simulink model "timedSpikingTestOpt2"  (R2026b)
settings: Solver=FixedStepAuto  StopTime=15  FixedStep=0.001
libraries: simulink x1, dspsigops x1
settings Model: Creator=40129232  LastModifiedBy=Eoin
settings DataIOCC: ReturnWorkspaceOutputs=off
settings OptimizationCC: LifeSpan=inf
settings DebuggingCC: ArithmeticOperatorsInVariantConditions=warning  SFExecutionAtInitializationDiag=none
settings SFSimCC: CustomCodeUndefinedFunction=UseInterfaceOnly  SimUseLocalCustomCode=off
settings RTWCC: DLArmComputeVersion=19.05  RTWUseLocalCustomCode=off
settings CodeAppCC: StateflowObjectComments=on

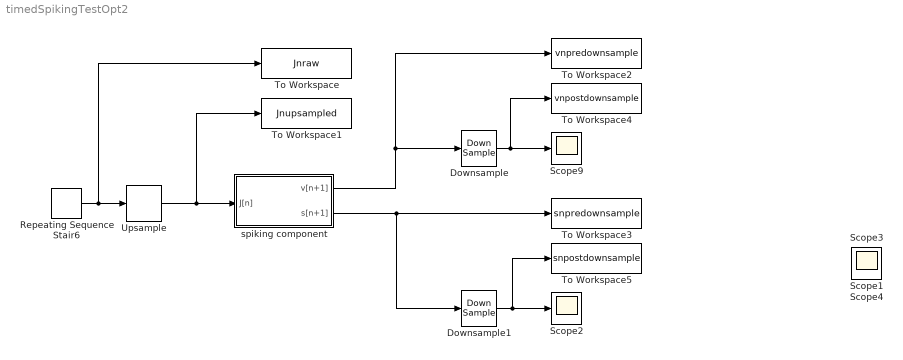
== system timedSpikingTestOpt2 ==
  Downsample : DownSample  DownsamplingFactor=15
  Downsample1 : DownSample  DownsamplingFactor=15
  Repeating Sequence Stair6 : simulink/Sources/Repeating Sequence Stair  OutValues=[40.37, 52.35, 62.17, 70.19, 76.75].'  tsamp=0.015  OutMin=[]  OutMax=[]  OutDataTypeStr=double  OutputDataTypeScalingMode=double  OutDataType=fixdt(0,8)  ConRadixGroup=Best Precision: Vector-wise  OutScaling=2^-12
  Scope{1..4,9} (5 alike) : Scope
      Scope2 settings: ActiveDisplayYMinimum=-0.36753410515202733  ActiveDisplayYMaximum=1.2278178479729731
      Scope9 settings: ActiveDisplayYMinimum=-91.1513790892599  ActiveDisplayYMaximum=42.518602095331268  DataLoggingVariableName=ScopeData5
      Scope1 settings: ActiveDisplayYMinimum=-0.24987  ActiveDisplayYMaximum=2.24887
      Scope3 settings: ActiveDisplayYMinimum=-103.72127  ActiveDisplayYMaximum=38.33358  DataLoggingVariableName=ScopeData3
      Scope4 settings: ActiveDisplayYMinimum=-20.75486  ActiveDisplayYMaximum=56.79378  DataLoggingVariableName=ScopeData4
  To Workspace : ToWorkspace  VariableName=Jnraw  SaveFormat=Timeseries  SampleTime=-1
  To Workspace1 : ToWorkspace  VariableName=Jnupsampled  SaveFormat=Timeseries  SampleTime=-1
  To Workspace2 : ToWorkspace  VariableName=vnpredownsample  SaveFormat=Timeseries  SampleTime=-1
  To Workspace3 : ToWorkspace  VariableName=snpredownsample  SaveFormat=Timeseries  SampleTime=-1
  To Workspace4 : ToWorkspace  VariableName=vnpostdownsample  SaveFormat=Timeseries  SampleTime=-1
  To Workspace5 : ToWorkspace  VariableName=snpostdownsample  SaveFormat=Timeseries  SampleTime=-1
  Upsample : dspsigops/Upsample  FactorSource=Dialog parameter  UpsamplingFactor=15  MaxUpsamplingFactor=100  SampleOffset=0  RateOptions=Allow multirate processing  InitialConditions=0  mode=Unused parameter value
      settings: LibrarySourceBlock=dsphdlsupportsigops/Upsample
  spiking component : Subsystem
  wires:
  Downsample/1 -> To Workspace4/1, Scope9/1
  Downsample1/1 -> To Workspace5/1, Scope2/1
  Repeating Sequence Stair6/1 -> To Workspace/1, Upsample/1
  spiking component/2(s[n+1]) -> To Workspace3/1, Downsample1/1
  spiking component/1(v[n+1]) -> To Workspace2/1, Downsample/1
  Upsample/1 -> spiking component/1(J[n]), To Workspace1/1

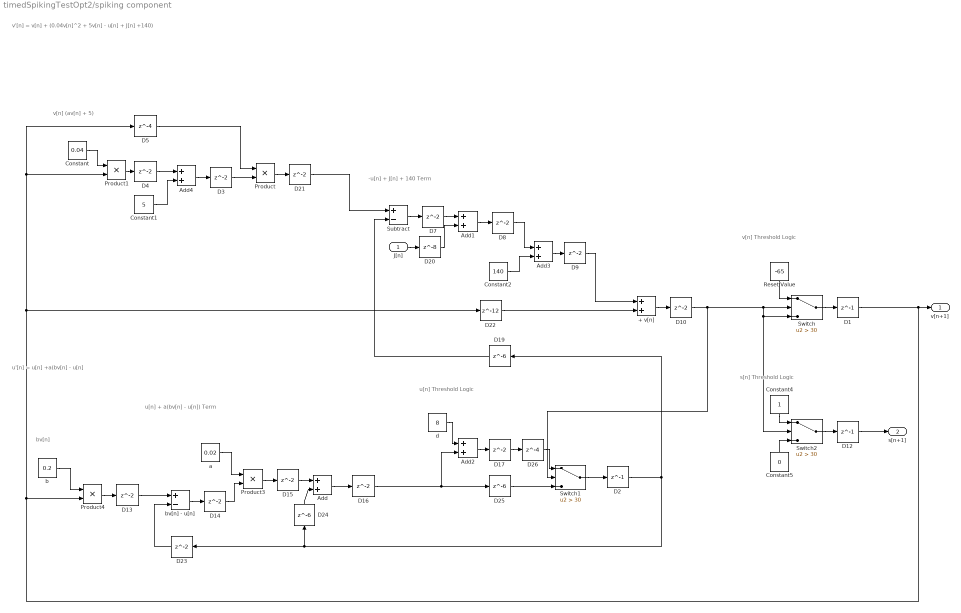
== system timedSpikingTestOpt2/spiking component ==
  note: v[n] (av[n] + 5)
  note: u'[n] = u[n] +a(bv[n] - u[n]
  note: s[n] Threshold Logic
  note: u[n] Threshold Logic
  note: u[n] + a(bv[n] - u[n]) Term
  note: -u[n] + J[n] + 140 Term
  note: v[n] Threshold Logic
  note: bv[n]
  note: v'[n] = v[n] + (0.04v[n]^2 + 5v[n] - u[n] + J[n] +140)
  J[n] : Inport  SampleTime=0.001
  + v[n] : Sum
  Add{,1..4} (5 alike) : Sum
  Constant : Constant  Value=0.04
  Constant1 : Constant  Value=5
  Constant2 : Constant  Value=140
  Constant4 : Constant
  Constant5 : Constant  Value=0
  D1 : Delay  DelayLength=1  InitialCondition=-65
  D{3..4,7..10,13..17,21,23} (13 alike) : Delay  InitialCondition=0
  D12 : Delay  DelayLength=1  InitialCondition=0
  D19 : Delay  DelayLength=6  InitialCondition=0
  D2 : Delay  DelayLength=1  InitialCondition=0
  D20 : Delay  DelayLength=8  InitialCondition=0
  D22 : Delay  DelayLength=12  InitialCondition=0
  D24 : Delay  DelayLength=6  InitialCondition=0
  D25 : Delay  DelayLength=6  InitialCondition=0
  D26 : Delay  DelayLength=4  InitialCondition=0
  D5 : Delay  DelayLength=4  InitialCondition=0
  Product{,1,3..4} (4 alike) : Product
  Reset Value : Constant  Value=-65
  Subtract : Sum  Inputs=+-
  Switch : Switch  Criteria=u2 > Threshold  Threshold=30  SaturateOnIntegerOverflow=off  InputSameDT=off
  Switch1 : Switch  Criteria=u2 > Threshold  Threshold=30  SaturateOnIntegerOverflow=off  InputSameDT=off
  Switch2 : Switch  Criteria=u2 > Threshold  Threshold=30  SaturateOnIntegerOverflow=off  InputSameDT=off
  a : Constant  Value=0.02
  b : Constant  Value=0.2
  bv[n] - u[n] : Sum  Inputs=+-
  d : Constant  Value=8
  v[n+1] : Outport  VectorParamsAs1DForOutWhenUnconnected=off
  s[n+1] : Outport  Port=2  VectorParamsAs1DForOutWhenUnconnected=off
  wires:
  Reset Value/1 -> Switch/1
  Constant1/1 -> Add4/2
  Constant5/1 -> Switch2/3
  d/1 -> Add2/1
  Constant4/1 -> Switch2/1
  b/1 -> Product4/1
  Constant2/1 -> Add3/2
  a/1 -> Product3/1
  Constant/1 -> Product1/1
  Subtract/1 -> D7/1
  Add3/1 -> D9/1
  Switch2/1 -> D12/1
  Product3/1 -> D15/1
  Add2/1 -> D17/1
  Product1/1 -> D4/1
  J[n]/1 -> D20/1
  Add/1 -> D16/1
  + v[n]/1 -> D10/1
  Product4/1 -> D13/1
  Product/1 -> D21/1
  D7/1 -> Add1/1
  Add1/1 -> D8/1
  D8/1 -> Add3/1
  D9/1 -> + v[n]/1
  D12/1 -> s[n+1]/1
  D13/1 -> bv[n] - u[n]/1
  bv[n] - u[n]/1 -> D14/1
  D14/1 -> Product3/2
  D16/1 -> D25/1, Add2/2
  D15/1 -> Add/1
  D19/1 -> Subtract/2
  D20/1 -> Add1/2
  D22/1 -> + v[n]/2
  D23/1 -> bv[n] - u[n]/2
  D24/1 -> Add/2
  D25/1 -> Switch1/3
  D17/1 -> D26/1
  D26/1 -> Switch1/1
  D10/1 -> Switch1/2, Switch/3, Switch2/2, Switch/2
  D21/1 -> Subtract/1
  Switch/1 -> D1/1
  Switch1/1 -> D2/1
  D4/1 -> Add4/1
  Add4/1 -> D3/1
  D3/1 -> Product/2
  D5/1 -> Product/1
  D1/1 -> Product4/2, D22/1, Product1/2, D5/1, v[n+1]/1
  D2/1 -> D19/1, D23/1, D24/1
